simulink model "commhdlQPSKTxRxLoopback"  (R2025b)
settings: Solver=FixedStepDiscrete  StartTime=0.0  StopTime=stopTime  RelTol=1e-3
PostLoadFcn:
  | hScopeConfig = get_param([gcs '/Receiver/QPSK Rx/Frequency and Time Synchronizer/Symbol Synchronizer/No HDL/QPSK Receiver Eye Diagram'],'ScopeConfiguration');
  | 
  | hScopeConfig.OpenAtSimulationStart = false;
  | hScopeConfig.Visible = false;
  | SamplesPerSymbol = 4;
  | %UpsamplesRx = 1;
  | clear hScopeConfig
InitFcn:
  | commhdlQPSKTxRxModelInit;
  | % Rate bridge: ADRV9002/Jupiter radio runs at 15.36 MHz = 2x the 7.68 MHz
  | % (4 samples/symbol @ Rsym=1.92 MHz) the QPSK Rx requires. The deployed
  | % Receiver must downsample the ADC stream by 2. UpsamplesRx=1 fed the QPSK
  | % Rx 8 sps (2x-upsampled) and broke symbol sync / the loopback bit check.
  | UpsamplesRx = 1;   %% T8 RATE FIX: rail 15.36e6 == ADC bus rate,
  | %% no ingress decimation (was 2 when the rail sat on the 7.68e6 rung)
  | UpsamplesTx = 1;
  | clear simTimingOffset;
StopFcn:
  | if exist('simTimingOffset','var')
  |   disp('Simulation completed');
  |   %QPSKTxRxVerification;
  | end
undefined symbols (not defined in the file or in its folder): Add, Config, fsym, randsrc, RandStream, Rsym, Shift
libraries: hdlsllib x141, simulink x43, dspsigops x34, dsphdlfiltering2 x6, dsphdlsigops2 x4, dsphdlmathfun2 x4, commdigbbndpm3 x4, dspmlti4 x2, commchan3 x1, commrflib2 x1, commcnvcod2 x1
(part 3 of 8)

== system commhdlQPSKTxRxLoopback/Receiver/QPSK Rx/Frequency and Time Synchronizer/Coarse Frequency Compensator ==
  dataIn : Inport
  validIn : Inport  Port=2
  CFO step change detector : Subsystem
  Coarse Frequency Estimator : Subsystem
  Data Type Conversion2 : DataTypeConversion  OutDataTypeStr=fixdt(1,16,12)  SaturateOnIntegerOverflow=off  RndMeth=Floor
  Data Type Conversion3 : DataTypeConversion  OutDataTypeStr=fixdt(1,21,21)  SaturateOnIntegerOverflow=off  RndMeth=Floor
  Data Type Conversion4 : DataTypeConversion  OutDataTypeStr=fixdt(1,21,0)  ConvertRealWorld=Stored Integer (SI)  SaturateOnIntegerOverflow=off  RndMeth=Floor
  Delay1 : Delay  DelayLength=9
  Delay{11..17} (7 alike) : Delay
  Delay2 : Delay  DelayLength=9
  Delay3 : Delay  DelayLength=6
  Delay4 : Delay  DelayLength=6
  Delay5 : Delay  DelayLength=1
  Delay6 : Delay  DelayLength=1
  Delay7 : Delay  DelayLength=12
  Delay8 : Delay  DelayLength=12
  Gain : Gain  Gain=1/4  ParamDataTypeStr=fixdt(0,2,2)  OutDataTypeStr=Inherit: Same as input
  Math Function : Math  Operator=conj
  NCO : dsphdlsigops2/NCO  PhaseIncrementSource=Input port  PhaseIncrement=100  PhaseOffsetSource=Property  PhaseOffset=0  DitherSource=None  NumDitherBits=4  SamplesPerFrame=1  LUTCompress=off  ResetAction=off  Waveform=Complex exponential  PhasePort=off  SimulateUsing=Code generation  AccumulatorWL=21  PhaseQuantization=on  NumQuantizerAccumulatorBits=14  OutputDataType=Binary point scaling  OutputWL=16  OutputFL=14
  Product1 : Product  OutDataTypeStr=Inherit: Same as first input
  Raise Power to 4 : Subsystem
  Terminator : Terminator
  dataOut : Outport
  rstCS : Outport  Port=2
  validOut : Outport  Port=3
  normalizedFreqEst : Outport  Port=4
  wires:
  Delay14/1 -> Delay15/1
  Delay11/1 -> Product1/1
  Delay6/1 -> Raise Power to 4/2(validIn), Delay2/1
  Delay5/1 -> Delay1/1, Data Type Conversion2/1
  Data Type Conversion4/1 -> NCO/1
  Delay4/1 -> Delay14/1
  Delay3/1 -> Delay11/1
  Delay2/1 -> Delay8/1
  Delay1/1 -> Delay7/1
  NCO/2 -> Terminator/1
  NCO/1 -> Math Function/1
  Product1/1 -> Delay13/1
  Raise Power to 4/2(validOut) -> Coarse Frequency Estimator/2(validIn)
  Math Function/1 -> Delay12/1
  Raise Power to 4/1(dataOut) -> Coarse Frequency Estimator/1(dataIn)
  Delay12/1 -> Product1/2
  Coarse Frequency Estimator/1(normFreqEst) -> Gain/1
  Data Type Conversion2/1 -> Raise Power to 4/1(dataIn)
  Delay16/1 -> Delay17/1
  CFO step change detector/1(Out1) -> Delay16/1
  Gain/1 -> Data Type Conversion3/1
  Delay13/1 -> dataOut/1
  dataIn/1 -> Delay5/1
  validIn/1 -> Delay6/1
  Delay17/1 -> rstCS/1
  Data Type Conversion3/1 -> normalizedFreqEst/1, CFO step change detector/1(In1), Data Type Conversion4/1
  Delay15/1 -> validOut/1
  Delay7/1 -> Delay3/1
  Delay8/1 -> NCO/2, Delay4/1

== system commhdlQPSKTxRxLoopback/Receiver/QPSK Rx/Frequency and Time Synchronizer/No HDL ==
  In1 : Inport
  In2 : Inport  Port=2
  In3 : Inport  Port=3
  In4 : Inport  Port=4
  Data Type Conversion : DataTypeConversion  OutDataTypeStr=double  SaturateOnIntegerOverflow=off  RndMeth=Floor
  Data Type Conversion1 : DataTypeConversion  OutDataTypeStr=double  SaturateOnIntegerOverflow=off  RndMeth=Floor
  QPSK Receiver Constellations 2 : ConstellationDiagram  NumInputPorts=2  WindowPosition=[67.000000,180.000000,973.000000,678.000000,]  Visible=on  ScopeFrameLocation=window  SymbolsToDisplaySource=Property  SymbolsToDisplay=10000  ReferenceConstellation="{[0.70711+0.70711i        -0.70711+0.70711i        -0.70711-0.70711i         0.70711-0.70711i],[0.70711+0.70711i        -0.70711+0.70711i        -0.70711-0.70711i         0.70711-0.70711i]}"  ReferenceMarker={''+'',''+''}  ReferenceColor={[1 0 0],[1 0 0]}  XLimits=[-1.3581 1.3569]  YLimits=[-1.3581 1.3569]  AxesLimits=[-1.3581 1.3569]  ShowLegend=on  DefaultConfigurationName=comm.scopes.ConstellationDiagramBlockCfg
      settings: OpenAtSimulationStart=off
  Subsystem : Subsystem
  Unit Delay Enabled Synchronous : hdlsllib/Discrete/Unit Delay Enabled Synchronous  InitialCondition=0.0  SampleTime=-1
  Unit Delay Enabled Synchronous1 : hdlsllib/Discrete/Unit Delay Enabled Synchronous  InitialCondition=0.0  SampleTime=-1
  wires:
  In4/1 -> Unit Delay Enabled Synchronous1/2, Subsystem/Enable
  Data Type Conversion/1 -> Unit Delay Enabled Synchronous1/1, Subsystem/1(In1)
  Unit Delay Enabled Synchronous1/1 -> QPSK Receiver Constellations 2/2  "After Carrier Synchronization"
  In2/1 -> Unit Delay Enabled Synchronous/2
  In1/1 -> Data Type Conversion1/1
  Data Type Conversion1/1 -> Unit Delay Enabled Synchronous/1
  Unit Delay Enabled Synchronous/1 -> QPSK Receiver Constellations 2/1  "After Symbol Synchronization"
  In3/1 -> Data Type Conversion/1

== system commhdlQPSKTxRxLoopback/Receiver/QPSK Rx/Frequency and Time Synchronizer/Packet Controller ==
  dataIn : Inport
  syncPulse : Inport  Port=2
  validIn : Inport  Port=3
  Delay : Delay  DelayLength=4
  Delay1 : Delay  DelayLength=4
  Delay2 : Delay  DelayLength=4
  End Generator : Subsystem
  Logical Operator : Logic  IconShape=distinctive  AllPortsSameDT=off  OutDataTypeStr=boolean
  MATLAB Function : MATLAB Function  TreatAsAtomicUnit=on
  Time Scope End Generator : Scope  Commented=on  NumInputPorts=2
      settings: SampleTime=1  ActiveDisplayYMinimum=-0.048155737704917989  ActiveDisplayYMaximum=1.0464480874316939  YLabel=Amplitude  DataLoggingVariableName=ScopeData2
  To File : ToFile  Filename=end_gen.mat  MatrixName=end_gen  SaveFormat=Timeseries
  To File1 : ToFile  Filename=reset  MatrixName=reset  SaveFormat=Timeseries
  sample discard controller : MATLAB Function  TreatAsAtomicUnit=on
  dataOut : Outport
  startOut : Outport  Port=2
  endOut : Outport  Port=3
  validOut : Outport  Port=4
  wires:
  MATLAB Function/1(out) -> Logical Operator/2
  sample discard controller/1(dataOut) -> dataOut/1
  sample discard controller/2(startOut) -> startOut/1
  sample discard controller/3(endOut) -> endOut/1
  sample discard controller/4(validOut) -> validOut/1
  Delay/1 -> sample discard controller/1(dataIn)
  Delay1/1 -> sample discard controller/2(validIn), End Generator/1(validIn)
  Delay2/1 -> sample discard controller/3(startIn)
  dataIn/1 -> Delay/1
  validIn/1 -> MATLAB Function/1(valid), Delay1/1, Logical Operator/1
  Logical Operator/1 -> Delay2/1, To File1/1, Time Scope End Generator/2, End Generator/2(rst)
  syncPulse/1 -> MATLAB Function/2(syncPulse)
  End Generator/1(endOut) -> Time Scope End Generator/1, To File/1, sample discard controller/4(endIn)

== system commhdlQPSKTxRxLoopback/Receiver/QPSK Rx/Frequency and Time Synchronizer/Phase Ambiguity Estimation and Correction ==
  dataIn : Inport
  syncPulseIn : Inport  Port=2
  validIn : Inport  Port=3
  Average Estimates : Subsystem
  Delay : Delay  DelayLength=32
  Delay1 : Delay  DelayLength=32
  Delay10 : Delay  DelayLength=15 + 7
  Delay11 : Delay  DelayLength=5
  Delay12 : Delay  DelayLength=5
  Delay13 : Delay  DelayLength=5
  Delay2 : Delay  DelayLength=32
  Delay3 : Delay  DelayLength=8
  Delay4 : Delay  DelayLength=8
  Delay5 : Delay  DelayLength=8
  Delay6 : Delay  DelayLength=1
  Delay7 : Delay  DelayLength=1
  Delay8 : Delay  DelayLength=1
  Delay9 : Delay  DelayLength=10
  Phase Ambiguity Corrector : Subsystem
  Phase Ambiguity Estimator : Subsystem
  dataOut : Outport
  syncPulseOut : Outport  Port=2
  validOut : Outport  Port=3
  wires:
  Delay4/1 -> Delay2/1
  Delay5/1 -> Delay/1
  Delay3/1 -> Delay1/1
  Delay10/1 -> Delay9/1
  Phase Ambiguity Corrector/1(dataOut) -> dataOut/1
  Phase Ambiguity Corrector/2(validOut) -> validOut/1
  Delay9/1 -> syncPulseOut/1
  Delay8/1 -> Phase Ambiguity Corrector/1(dataIn)
  Average Estimates/1(avgEst) -> Phase Ambiguity Corrector/2(estimate)
  Delay7/1 -> Phase Ambiguity Corrector/3(validIn)
  Delay6/1 -> Delay10/1
  dataIn/1 -> Delay5/1
  validIn/1 -> Delay4/1
  Delay13/1 -> Delay8/1
  Phase Ambiguity Estimator/1(endOut) -> Average Estimates/1(endIn)
  Phase Ambiguity Estimator/3(validOut) -> Average Estimates/3(validIn)
  Delay12/1 -> Delay7/1
  Delay11/1 -> Delay6/1
  Phase Ambiguity Estimator/2(estOut) -> Average Estimates/2(estin)
  Delay/1 -> Delay13/1, Phase Ambiguity Estimator/1(dataIn)
  syncPulseIn/1 -> Phase Ambiguity Estimator/2(syncPulse), Delay3/1
  Delay2/1 -> Phase Ambiguity Estimator/3(validIn), Delay12/1
  Delay1/1 -> Delay11/1

== system commhdlQPSKTxRxLoopback/Receiver/QPSK Rx/Frequency and Time Synchronizer/Preamble Detector ==
  dataIn : Inport
  validIn : Inport  Port=2
  Constant : Constant  Value=false  SampleTime=-1
  Correlator : Subsystem
  Delay : Delay  DelayLength=20
  Delay{1..5,11..14} (9 alike) : Delay  DelayLength=1
  Delay10 : Delay  DelayLength=searchSamples * 4
  Delay6 : Delay  DelayLength=6
  Delay7 : Delay  DelayLength=20
  Delay8 : Delay  DelayLength=6
  FIFO : Subsystem  mask{fifoSize=searchSamples, pushFullDiag=Error, popEmptyDiag=Error}
      mask prompts: fifoSize "FIFO size:"; pushFullDiag "Push full FIFO:"; popEmptyDiag "Pop empty FIFO:"
      mask TypeOptions pushFullDiag: Ignore | Warning | Error
      mask TypeOptions popEmptyDiag: Ignore | Warning | Error
  Logical Operator : Logic  AllPortsSameDT=off  OutDataTypeStr=boolean
  No HDL : Subsystem
  Peak Search : Subsystem  VariantControl=new  mask{samplesPerFrame=searchSamples}
      mask prompts: samplesPerFrame "Number of samples to search:"
      mask init:
      | samplesPerFrame1x            = samplesPerFrame;
      |     searchDuration               = samplesPerFrame1x;
  Relational Operator : RelationalOperator  Operator=>  OutDataTypeStr=boolean  InputSameDT=off
  Terminator : Terminator
  Terminator1 : Terminator
  Timing Adjust : Subsystem
  dataOut : Outport
  syncPulse : Outport  Port=2
  validOut : Outport  Port=3
  wires:
  Delay/1 -> Delay6/1
  validIn/1 -> Delay2/1
  dataIn/1 -> Delay1/1
  Relational Operator/1 -> Peak Search/2(thresholdExceeded)
  Peak Search/3(success) -> Logical Operator/2  "success"
  Peak Search/2(done) -> Logical Operator/1  "done"
  Delay7/1 -> Delay8/1
  Timing Adjust/1(dataOut) -> Delay3/1  "synchronizedData"
  Timing Adjust/3(SyncPulse) -> Delay4/1  "synchronizedPulse"
  Timing Adjust/2(validOut) -> Delay5/1  "synchronizedValid"
  Delay3/1 -> dataOut/1
  Delay5/1 -> validOut/1
  Delay4/1 -> syncPulse/1
  Peak Search/1(timingOffset) -> Delay11/1
  Logical Operator/1 -> Delay12/1
  Delay10/1 -> FIFO/3(pop), Delay14/1
  Correlator/3(validOut) -> Peak Search/3(validIn), No HDL/Enable
  Correlator/2(threshold) -> Relational Operator/2, No HDL/2(In2)
  Correlator/1(dataOut) -> Relational Operator/1, Peak Search/1(corr), No HDL/1(In1)
  Delay8/1 -> FIFO/2(push), Delay10/1
  Delay1/1 -> Delay/1, Correlator/1(dataIn)
  Delay2/1 -> Delay7/1, Correlator/2(validIn)
  Delay11/1 -> Timing Adjust/1(timingOffset)
  Delay12/1 -> Timing Adjust/2(timingOffsetValid)
  Delay13/1 -> Timing Adjust/3(dataIn)
  Delay14/1 -> Timing Adjust/4(validIn)
  FIFO/2(numEntries) -> Terminator/1
  Constant/1 -> FIFO/4(reset)
  FIFO/3(validPop) -> Terminator1/1
  Delay6/1 -> FIFO/1(in)
  FIFO/1(out) -> Delay13/1

== system commhdlQPSKTxRxLoopback/Receiver/QPSK Rx/Frequency and Time Synchronizer/Symbol Synchronizer ==
  dataIn : Inport
  validIn : Inport  Port=2
  Data Type Conversion4 : DataTypeConversion  OutDataTypeStr=fixdt(1,16,14)  SaturateOnIntegerOverflow=off  RndMeth=Floor
  Delay{1..4,6,8..9} (7 alike) : Delay  DelayLength=1
  Delay5 : Delay  DelayLength=12
  Delay7 : Delay  DelayLength=12
  Gardner TED : Subsystem
  Integer Delay{1..4} (4 alike) : Delay  DelayLength=1
  Interpolation Control : MATLAB Function
  Interpolation Filter : Subsystem
  Loop Filter : Subsystem
  No HDL : Subsystem
  Rate Handle : Subsystem
  dataOut : Outport
  validOut : Outport  Port=2
  wires:
  Loop Filter/1(v) -> Delay4/1
  Gardner TED/1(e) -> Delay3/1
  Interpolation Control/2(Underflow) -> Integer Delay3/1
  Integer Delay4/1 -> Interpolation Filter/2(mu)
  dataIn/1 -> No HDL/1(data), Integer Delay1/1
  Integer Delay3/1 -> Delay5/1
  Delay3/1 -> Loop Filter/1(e)
  Delay4/1 -> Interpolation Control/1(Delta)
  Data Type Conversion4/1 -> Rate Handle/1(dataIn)
  Delay1/1 -> Data Type Conversion4/1
  Delay6/1 -> Rate Handle/3(validIn)
  Delay7/1 -> Delay6/1
  validIn/1 -> No HDL/2(valid), Integer Delay2/1
  Rate Handle/2(validOut) -> validOut/1
  Rate Handle/1(dataOut) -> dataOut/1
  Interpolation Filter/1(interpolant) -> Delay8/1, Delay1/1
  Interpolation Control/1(mu) -> Integer Delay4/1
  Delay2/1 -> Rate Handle/2(strobe)
  Delay5/1 -> Delay9/1, Delay2/1
  Integer Delay1/1 -> Interpolation Filter/1(In)
  Integer Delay2/1 -> Delay7/1
  Delay8/1 -> Gardner TED/1(data)
  Delay9/1 -> Gardner TED/2(strobe)

== system commhdlQPSKTxRxLoopback/Receiver/QPSK Rx/QPSK Demodulator/Serializer ==
  u : Inport
  In2 : Inport  Port=2
  Delay1 : Delay  DelayLength=1
  Delay4 : Delay  DelayLength=1
  Demux : Demux  Outputs=2
  HDL Counter : hdlsllib/Sources/HDL Counter  CountType=Count limited  CountInit=0  CountStep=1  CountMax=1  CountFromType=Initial value  CountFrom=0  CountResetPort=off  CountLoadPort=off  CountEnbPort=on  CountDirPort=off  CountHitOutputPort=off  CountDataType=Unsigned  CountWordLen=1  CountFracLen=0  CountSampTime=1
  Logical Operator : Logic  Operator=OR  AllPortsSameDT=off  OutDataTypeStr=boolean
  Multiport Switch : MultiPortSwitch  DataPortOrder=Zero-based contiguous  Inputs=2  zeroidx=on  SaturateOnIntegerOverflow=off  InputSameDT=off
  Unit Delay Enabled Synchronous : hdlsllib/Discrete/Unit Delay Enabled Synchronous  InitialCondition=0.0  SampleTime=-1
  Out1 : Outport
  Out2 : Outport  Port=2
  wires:
  Demux/2 -> Multiport Switch/3
  Logical Operator/1 -> Out2/1, HDL Counter/1
  In2/1 -> Unit Delay Enabled Synchronous/2, Delay1/1
  HDL Counter/1 -> Multiport Switch/1
  Delay4/1 -> Logical Operator/2
  u/1 -> Unit Delay Enabled Synchronous/1
  Multiport Switch/1 -> Out1/1
  Demux/1 -> Multiport Switch/2
  Delay1/1 -> Logical Operator/1, Delay4/1
  Unit Delay Enabled Synchronous/1 -> Demux/1

== system commhdlQPSKTxRxLoopback/Transmitter/QPSK Tx/Bit Packetizer/Data Bits FIFO ==
  data : Inport
  push : Inport  Port=2
  Compare To Constant : simulink/Logic and Bit Operations/Compare To Constant  relop=>=  const=length(Preamble)  OutDataTypeStr=boolean
  Compare To Constant1 : simulink/Logic and Bit Operations/Compare To Constant  relop===  const=0  OutDataTypeStr=boolean
  Compare To Constant2 : simulink/Logic and Bit Operations/Compare To Constant  relop=~=  const=0  OutDataTypeStr=boolean
  Compare To Constant3 : simulink/Logic and Bit Operations/Compare To Constant  relop===  const=0  OutDataTypeStr=boolean
  Compare To Constant4 : simulink/Logic and Bit Operations/Compare To Constant  relop===  const=bitsPerPacket - 1  OutDataTypeStr=boolean
  Compare To Constant5 : hdlsllib/Logic and Bit Operations/Compare To Constant  relop===  const=Config.SamplesPerSymbol/2 -1  OutDataTypeStr=boolean
  Constant : Constant  Value=true  SampleTime=1/(Rsym*SamplesPerSymbol)
  Delay{1..7} (7 alike) : Delay  DelayLength=1
  HDL Counter : hdlsllib/Sources/HDL Counter  CountType=Count limited  CountInit=0  CountStep=1  CountMax=dataBitsPerPacket*2 - 1  CountFromType=Initial value  CountFrom=0  CountResetPort=off  CountLoadPort=off  CountEnbPort=on  CountDirPort=off  CountHitOutputPort=off  CountDataType=Unsigned  CountWordLen=nextpow2(dataBitsPerPacket*2 - 1)  CountFracLen=0  CountSampTime=1
  HDL Counter1 : hdlsllib/Sources/HDL Counter  CountType=Count limited  CountInit=0  CountStep=1  CountMax=dataBitsPerPacket*2 - 1  CountFromType=Initial value  CountFrom=0  CountResetPort=off  CountLoadPort=off  CountEnbPort=on  CountDirPort=off  CountHitOutputPort=off  CountDataType=Unsigned  CountWordLen=nextpow2(dataBitsPerPacket*2 - 1)  CountFracLen=0  CountSampTime=1
  HDL Counter2 : hdlsllib/Sources/HDL Counter  CountType=Count limited  CountInit=0  CountStep=1  CountMax=bitsPerPacket - 1  CountFromType=Initial value  CountFrom=0  CountResetPort=off  CountLoadPort=off  CountEnbPort=on  CountDirPort=off  CountHitOutputPort=off  CountDataType=Unsigned  CountWordLen=nextpow2(bitsPerPacket)  CountFracLen=0  CountSampTime=1
  HDL Counter3 : hdlsllib/Sources/HDL Counter  CountType=Count limited  CountInit=0  CountStep=1  CountMax=Config.SamplesPerSymbol/2 -1  CountFromType=Initial value  CountFrom=0  CountResetPort=off  CountLoadPort=off  CountEnbPort=on  CountDirPort=off  CountHitOutputPort=off  CountDataType=Unsigned  CountWordLen=nextpow2(Config.SamplesPerSymbol/2)  CountFracLen=0  CountSampTime=1
  Logical Operator : Logic  Inputs=3  AllPortsSameDT=off  OutDataTypeStr=boolean
  Logical Operator1 : Logic  Inputs=3  AllPortsSameDT=off  OutDataTypeStr=boolean
  MATLAB Function1 : MATLAB Function  TreatAsAtomicUnit=on
  No HDL : Subsystem
  RAM Frame Status Indicator : MATLAB Function  TreatAsAtomicUnit=on
  Simple Dual Port RAM : hdlsllib/HDL RAMs/Simple Dual Port RAM  ram_size=nextpow2(dataBitsPerPacket*2 - 1)
  Unit Delay Enabled Resettable Synchronous : hdlsllib/Discrete/Unit Delay Enabled Resettable Synchronous  InitialCondition=0.0  SampleTime=-1
  dataOut : Outport
  activeFrame : Outport  Port=2
  sampleCount : Outport  Port=3
  sampleCountValid : Outport  Port=4
  fullRAM : Outport  Port=5
  wires:
  HDL Counter1/1 -> Simple Dual Port RAM/4
  HDL Counter/1 -> Simple Dual Port RAM/2
  data/1 -> Simple Dual Port RAM/1
  Constant/1 -> HDL Counter3/1
  HDL Counter2/1 -> Compare To Constant/1, Delay2/1, Compare To Constant3/1
  Compare To Constant1/1 -> Unit Delay Enabled Resettable Synchronous/3
  RAM Frame Status Indicator/1(out) -> Delay3/1
  Compare To Constant2/1 -> Logical Operator1/1, Unit Delay Enabled Resettable Synchronous/1
  Compare To Constant3/1 -> Unit Delay Enabled Resettable Synchronous/2
  Compare To Constant/1 -> Delay1/1
  Delay1/1 -> Logical Operator/2
  Delay2/1 -> Delay5/1
  Delay3/1 -> Compare To Constant2/1, Compare To Constant1/1
  Simple Dual Port RAM/1 -> dataOut/1
  Delay4/1 -> Logical Operator/3, Delay6/1
  Delay5/1 -> Compare To Constant4/1, sampleCount/1
  Delay6/1 -> Logical Operator1/3, sampleCountValid/1
  Unit Delay Enabled Resettable Synchronous/1 -> Logical Operator/1
  Compare To Constant4/1 -> Logical Operator1/2
  Logical Operator1/1 -> activeFrame/1
  Logical Operator/1 -> RAM Frame Status Indicator/2(pop), MATLAB Function1/2(rd), No HDL/2(pop), HDL Counter1/1
  push/1 -> MATLAB Function1/1(wr), RAM Frame Status Indicator/1(push), No HDL/1(push), HDL Counter/1, Simple Dual Port RAM/3
  MATLAB Function1/1(full) -> Delay7/1
  Delay7/1 -> fullRAM/1
  HDL Counter3/1 -> Compare To Constant5/1
  Compare To Constant5/1 -> HDL Counter2/1, Delay4/1

== system commhdlQPSKTxRxLoopback/Transmitter/QPSK Tx/Bit Packetizer/Preamble Bits Generator ==
  activeFrame : Inport
  sampleCount : Inport  Port=2
  sampleCountValid : Inport  Port=3
  Compare To Constant2 : hdlsllib/Logic and Bit Operations/Compare To Constant  relop===  const=bitsPerPacket - 1  OutDataTypeStr=boolean
  Logical Operator3 : Logic  AllPortsSameDT=off  OutDataTypeStr=boolean
  Preamble Bits Store : Subsystem
  Unit Delay Enabled Synchronous : hdlsllib/Discrete/Unit Delay Enabled Synchronous  InitialCondition=0.0  SampleTime=-1
  preambleBits : Outport
  wires:
  sampleCount/1 -> Compare To Constant2/1, Preamble Bits Store/2(sampleCount)
  Logical Operator3/1 -> Unit Delay Enabled Synchronous/2
  Preamble Bits Store/1(preamble) -> preambleBits/1
  Compare To Constant2/1 -> Logical Operator3/1
  Unit Delay Enabled Synchronous/1 -> Preamble Bits Store/1(actualPreamble)
  sampleCountValid/1 -> Logical Operator3/2
  activeFrame/1 -> Unit Delay Enabled Synchronous/1

== system commhdlQPSKTxRxLoopback/TxRxComposite/Receiver/QPSK Rx/Automatic Gain Control ==
  dataIn : Inport
  validIn : Inport  Port=2
  agc_loop_gain : Inport  Port=3  OutDataTypeStr=uint32  SampleTime=1/(Rsym*SamplesPerSymbol)
  Data Type Conversion : DataTypeConversion  OutDataTypeStr=fixdt(1,16,10)  SaturateOnIntegerOverflow=off  RndMeth=Floor
  Delay{1..5} (5 alike) : Delay
  Error Detector : Subsystem
  Loop Filter : Subsystem
  Product : Product  OutDataTypeStr=Inherit: Same as first input
  dataOut : Outport
  validOut : Outport  Port=2
  wires:
  Product/1 -> Delay2/1
  dataIn/1 -> Delay4/1
  Delay2/1 -> dataOut/1, Error Detector/1(dataIn)
  validIn/1 -> Delay5/1
  Error Detector/1(err) -> Loop Filter/1(err)
  Loop Filter/1(gain) -> Data Type Conversion/1
  Delay1/1 -> Product/2
  Delay4/1 -> Product/1
  Delay3/1 -> validOut/1
  Delay5/1 -> Delay3/1
  Data Type Conversion/1 -> Delay1/1
  agc_loop_gain/1 -> Loop Filter/2(agc_loop_gain)

== system commhdlQPSKTxRxLoopback/TxRxComposite/Receiver/QPSK Rx/FEC Decoder Wrapper ==
  bitsIn : Inport
  startIn : Inport  Port=2
  endIn : Inport  Port=3
  validIn : Inport  Port=4
  skipCount : Inport  Port=5  OutDataTypeStr=uint32  SampleTime=1/(Rsym*SamplesPerSymbol)
  FecCapture : MATLAB Function  TreatAsAtomicUnit=on
  FecCounters : MATLAB Function  TreatAsAtomicUnit=on
  RxAlign : MATLAB Function  TreatAsAtomicUnit=on
  RxDeint : MATLAB Function  TreatAsAtomicUnit=on
  VitGate : Subsystem
  dataOut : Outport
  startOut : Outport  Port=2
  endOut : Outport  Port=3
  validOut : Outport  Port=4
  cnt_descr_in : Outport  Port=5
  cnt_frame_start : Outport  Port=6
  cnt_vit_reset : Outport  Port=7
  cnt_deint_valid : Outport  Port=8
  cnt_dec_bits : Outport  Port=9
  cnt_bist_start : Outport  Port=10
  cap_in : Outport  Port=11
  cap_deint : Outport  Port=12
  cap_out : Outport  Port=13
  wires:
  bitsIn/1 -> RxDeint/1(dataIn), FecCapture/1(bitsIn)
  startIn/1 -> RxDeint/2(startIn), FecCounters/2(e2), FecCapture/3(startIn)
  endIn/1 -> RxDeint/3(endIn)
  validIn/1 -> RxDeint/4(validIn), FecCounters/1(e1), FecCapture/2(validIn)
  RxDeint/1(codedPair) -> VitGate/1(pairIn), FecCapture/4(codedPair)
  RxDeint/2(vitReset) -> VitGate/2(rstIn), FecCounters/3(e3)
  RxDeint/3(deintValid) -> VitGate/Enable, RxAlign/2(deintValid), FecCounters/4(e4), FecCapture/5(deintValid)
  VitGate/1(decOut) -> RxAlign/1(decBit)
  RxDeint/4(frameStart) -> RxAlign/3(frameStart)
  RxDeint/5(frameEnd) -> RxAlign/4(frameEnd)
  skipCount/1 -> RxAlign/5(skipCount), FecCapture/7(skipCount)
  RxAlign/1(dataOut) -> dataOut/1, FecCapture/6(decBit)
  RxAlign/2(startOut) -> startOut/1, FecCounters/6(e6)
  RxAlign/3(endOut) -> endOut/1
  RxAlign/4(validOut) -> validOut/1, FecCounters/5(e5), FecCapture/8(outValid)
  FecCounters/1(c1) -> cnt_descr_in/1
  FecCounters/2(c2) -> cnt_frame_start/1
  FecCounters/3(c3) -> cnt_vit_reset/1
  FecCounters/4(c4) -> cnt_deint_valid/1
  FecCounters/5(c5) -> cnt_dec_bits/1
  FecCounters/6(c6) -> cnt_bist_start/1
  FecCapture/1(capIn) -> cap_in/1
  FecCapture/2(capDeint) -> cap_deint/1
  FecCapture/3(capOut) -> cap_out/1

== system commhdlQPSKTxRxLoopback/TxRxComposite/Receiver/QPSK Rx/Frequency and Time Synchronizer ==
  dataIn : Inport
  validIn : Inport  Port=2
  rstCS : Inport  Port=3
  cs_prop_gain : Inport  Port=4  OutDataTypeStr=uint32  SampleTime=1/(Rsym*SamplesPerSymbol)
  cs_integ_gain : Inport  Port=5  OutDataTypeStr=uint32  SampleTime=1/(Rsym*SamplesPerSymbol)
  ss_prop_gain : Inport  Port=6  OutDataTypeStr=uint32  SampleTime=1/(Rsym*SamplesPerSymbol)
  ss_integ_gain : Inport  Port=7  OutDataTypeStr=uint32  SampleTime=1/(Rsym*SamplesPerSymbol)
  cfo_threshold : Inport  Port=8  OutDataTypeStr=uint32  SampleTime=1/(Rsym*SamplesPerSymbol)
  Carrier Synchronizer : Subsystem
      settings: PortSchema="{\"entries\":[{\"content\":{\"sides\":[{\"content\":{\"connectorIds\":[\"In1\",\"In2\",\"In3\"]},\"type\":\"ConnectorPlacement.EquallySpacedRectSide\",\"uuid\":\"ee58e5dc-083a-48cb-b7f3-66ed8a15890f\"},{\"content\":{\"connectorIds\":[\"Out1\",\"Out2\"],\"side\":\"RIGHT\"},\"type\":\"ConnectorPlacement.EquallySpacedRectSide\",\"uuid\":\"6d121164-5065-4840-a82e-fa57a8e9650e\"},{\"content\":{\"connectorIds\":[\"In4\",\"In5\",\"In6\"],\"side\":\"TOP\"},\"type\":\"ConnectorPlacement.EquallySpacedRectSide\",\"uuid\":\"54d2b8e3-f516-4572-94a0-c914196ae8e4\"}]},\"type\":\"ConnectorPlacement.EquallySpacedConnector\",\"uuid\":\"0f2a6472-efd0-42ca-a030-ab436081b5e1\"}],\"packageUris\":[\"http://schema.mathworks.com/mf0/Connector/R2020b\"],\"version\":\"1.0\"}"
  Coarse Frequency Compensator : Subsystem
      settings: PortSchema="{\"entries\":[{\"content\":{\"sides\":[{\"content\":{\"connectorIds\":[\"In1\",\"In2\",\"In3\"]},\"type\":\"ConnectorPlacement.EquallySpacedRectSide\",\"uuid\":\"138aa5bd-62db-47d6-b55f-f529a6004434\"},{\"content\":{\"connectorIds\":[\"Out1\",\"Out2\",\"Out3\"],\"side\":\"RIGHT\"},\"type\":\"ConnectorPlacement.EquallySpacedRectSide\",\"uuid\":\"8e6ccec0-f736-48ab-be6d-feac886e083d\"},{\"content\":{\"connectorIds\":[\"Out4\"],\"side\":\"TOP\"},\"type\":\"ConnectorPlacement.EquallySpacedRectSide\",\"uuid\":\"d4535392-74fa-432a-a39c-b98ba26e8163\"},{\"content\":{\"side\":\"BOTTOM\"},\"type\":\"ConnectorPlacement.EquallySpacedRectSide\",\"uuid\":\"770ac6a2-7a02-4a77-858b-592982deaf6e\"}]},\"type\":\"ConnectorPlacement.EquallySpacedConnector\",\"uuid\":\"a9b944be-f88b-4ab6-a5e1-6824362eb9ca\"}],\"packageUris\":[\"http://schema.mathworks.com/mf0/Connector/R2020b\"],\"version\":\"1.0\"}"
  No HDL : Subsystem
      settings: PortSchema="{\"entries\":[{\"content\":{\"sides\":[{\"content\":{\"connectorIds\":[\"In1\",\"In2\"]},\"type\":\"ConnectorPlacement.EquallySpacedRectSide\",\"uuid\":\"df96a46d-149f-4580-adf6-e5cf26cffa9b\"},{\"content\":{\"connectorIds\":[\"In3\",\"In4\"],\"side\":\"RIGHT\"},\"type\":\"ConnectorPlacement.EquallySpacedRectSide\",\"uuid\":\"1c46d09c-cb37-4618-ac4e-e5ef50df41fb\"},{\"content\":{\"connectorIds\":[],\"side\":\"TOP\"},\"type\":\"ConnectorPlacement.EquallySpacedRectSide\",\"uuid\":\"7fe62300-46d7-4234-a31d-eecffed4f6e6\"},{\"content\":{\"connectorIds\":[],\"side\":\"BOTTOM\"},\"type\":\"ConnectorPlacement.EquallySpacedRectSide\",\"uuid\":\"05ecd563-28f5-4cfd-b718-5032a7458763\"}]},\"type\":\"ConnectorPlacement.EquallySpacedConnector\",\"uuid\":\"4b3d5859-a469-4389-9e5d-e5f07416a9a1\"}],\"packageUris\":[\"http://schema.mathworks.com/mf0/Connector/R2020b\"],\"version\":\"1.0\"}"
  Packet Controller : Subsystem
  Phase Ambiguity Estimation and Correction : Subsystem
  Preamble Detector : Subsystem
  Symbol Synchronizer : Subsystem
  dataOut : Outport
  startOut : Outport  Port=2
  endOut : Outport  Port=3
  validOut : Outport  Port=4
  postSymbolSync : Outport  Port=5
  postCarrierSync : Outport  Port=6
  nSynced : Outport  Port=7
  normCoarseFreqEst : Outport  Port=8
  rstcsDet : Outport  Port=9
  p1c_telI : Outport  Port=10
  p1c_telQ : Outport  Port=11
  fs_runmax : Outport  Port=12
  wires:
  rstCS/1 -> Carrier Synchronizer/4(manualRst)
  Coarse Frequency Compensator/4(normalizedFreqEst) -> normCoarseFreqEst/1
  Carrier Synchronizer/2(validOut) -> Preamble Detector/2(validIn), No HDL/4(In4)
  Carrier Synchronizer/1(dataOut) -> Preamble Detector/1(dataIn), No HDL/3(In3), postCarrierSync/1
  Preamble Detector/2(syncPulse) -> Phase Ambiguity Estimation and Correction/2(syncPulseIn), nSynced/1
  Packet Controller/4(validOut) -> validOut/1
  Packet Controller/3(endOut) -> endOut/1
  Packet Controller/2(startOut) -> startOut/1
  Packet Controller/1(dataOut) -> dataOut/1
  Coarse Frequency Compensator/2(rstCS) -> Carrier Synchronizer/2(internalRst), rstcsDet/1
  dataIn/1 -> Symbol Synchronizer/1(dataIn)
  validIn/1 -> Symbol Synchronizer/2(validIn)
  Preamble Detector/1(dataOut) -> Phase Ambiguity Estimation and Correction/1(dataIn)
  Preamble Detector/3(validOut) -> Phase Ambiguity Estimation and Correction/3(validIn)
  Phase Ambiguity Estimation and Correction/2(syncPulseOut) -> Packet Controller/2(syncPulse)
  Symbol Synchronizer/1(dataOut) -> Coarse Frequency Compensator/1(dataIn), No HDL/1(In1), postSymbolSync/1
  Symbol Synchronizer/2(validOut) -> Coarse Frequency Compensator/2(validIn), No HDL/2(In2)
  Phase Ambiguity Estimation and Correction/3(validOut) -> Packet Controller/3(validIn)
  Phase Ambiguity Estimation and Correction/1(dataOut) -> Packet Controller/1(dataIn)
  Coarse Frequency Compensator/1(dataOut) -> Carrier Synchronizer/1(dataIn)
  Coarse Frequency Compensator/3(validOut) -> Carrier Synchronizer/3(validIn)
  Preamble Detector/4(p1c_telI) -> p1c_telI/1
  Preamble Detector/5(p1c_telQ) -> p1c_telQ/1
  cs_prop_gain/1 -> Carrier Synchronizer/5(cs_prop_gain)
  cs_integ_gain/1 -> Carrier Synchronizer/6(cs_integ_gain)
  ss_prop_gain/1 -> Symbol Synchronizer/3(ss_prop_gain)
  ss_integ_gain/1 -> Symbol Synchronizer/4(ss_integ_gain)
  cfo_threshold/1 -> Coarse Frequency Compensator/3(cfo_threshold)
  Preamble Detector/6(fs_runmax) -> fs_runmax/1

== system commhdlQPSKTxRxLoopback/TxRxComposite/Receiver/QPSK Rx/QPSK Demodulator ==
  dataIn : Inport
  startIn : Inport  Port=2
  endIn : Inport  Port=3
  validIn : Inport  Port=4
  Delay{,1..13} (14 alike) : Delay  DelayLength=1
  QPSK Demodulator Baseband : commdigbbndpm3/QPSK Demodulator Baseband  OutType=Bit  DecType=Hard decision  VarSource=Dialog  Variance=1  Dec=Gray  Ph=pi/4  outDtype1=boolean  outDtype2=Inherit via internal rule  derotateFactorWordLen=16  derotateFactorDataTypeStr=Inherit: Same word length as input  derotateFactorLastDataTypeStr=Inherit: Same word length as input
  Serializer : Subsystem
  Signal Specification : SignalSpecification  Dimensions=1
  dataOut : Outport
  startOut : Outport  Port=2
  endOut : Outport  Port=3
  validOut : Outport  Port=4
  wires:
  endIn/1 -> Delay3/1
  startIn/1 -> Delay2/1
  validIn/1 -> Delay1/1
  dataIn/1 -> Signal Specification/1
  Serializer/2(Out2) -> Delay9/1
  Serializer/1(Out1) -> Delay8/1
  Delay13/1 -> Delay11/1
  Delay4/1 -> Delay10/1
  Delay12/1 -> Serializer/1(u)
  Delay5/1 -> Serializer/2(In2)
  Delay11/1 -> endOut/1
  Delay10/1 -> startOut/1
  Delay9/1 -> validOut/1
  Delay8/1 -> dataOut/1
  QPSK Demodulator Baseband/1 -> Delay12/1
  Signal Specification/1 -> Delay/1
  Delay3/1 -> Delay7/1
  Delay2/1 -> Delay6/1
  Delay7/1 -> Delay13/1
  Delay6/1 -> Delay4/1
  Delay1/1 -> Delay5/1
  Delay/1 -> QPSK Demodulator Baseband/1

== system commhdlQPSKTxRxLoopback/TxRxComposite/Transmitter/Input Data/FEC Tx Encoder K5 ==
  bitIn : Inport
  enable : Inport  Port=2
  reset : Inport  Port=3
  start : Inport  Port=4
  ConvEncK5 : MATLAB Function  TreatAsAtomicUnit=on
  TxGateK5 : MATLAB Function  TreatAsAtomicUnit=on
  TxInterleaveK5 : MATLAB Function  TreatAsAtomicUnit=on
  encBit : Outport
  wires:
  bitIn/1 -> TxGateK5/1(bitIn)
  enable/1 -> TxGateK5/2(enable)
  reset/1 -> TxGateK5/3(reset)
  start/1 -> TxGateK5/4(start)
  TxGateK5/1(infoBit) -> ConvEncK5/1(infoBit)
  TxGateK5/2(encReset) -> ConvEncK5/2(encReset)
  TxGateK5/3(infoValid) -> ConvEncK5/3(infoValid), TxInterleaveK5/2(infoValid)
  ConvEncK5/1(codedPair) -> TxInterleaveK5/1(codedPair)
  TxGateK5/4(beatIdx) -> TxInterleaveK5/3(beatIdx)
  TxGateK5/5(frameValid) -> TxInterleaveK5/4(frameValid)
  TxGateK5/6(frameStart) -> TxInterleaveK5/5(frameStart)
  TxInterleaveK5/1(dataOut) -> encBit/1

== system commhdlQPSKTxRxLoopback/TxRxComposite/Transmitter/Input Data/Message Generator ==
  reset : Inport
  enable : Inport  Port=2
  MATLAB Function : MATLAB Function  TreatAsAtomicUnit=on
  out : Outport
  stop : Outport  Port=2
  start : Outport  Port=3
  valid : Outport  Port=4
  count : Outport  Port=5
  msg_count_out : Outport  Port=6
  wires:
  MATLAB Function/6(msg_count_out) -> msg_count_out/1
  MATLAB Function/5(count_out) -> count/1
  MATLAB Function/4(valid) -> valid/1
  enable/1 -> MATLAB Function/1(enable)
  MATLAB Function/2(start) -> start/1
  reset/1 -> MATLAB Function/2(reset)
  MATLAB Function/1(out) -> out/1
  MATLAB Function/3(stop) -> stop/1

== system commhdlQPSKTxRxLoopback/TxRxComposite/Transmitter/QPSK Tx/Bit Packetizer ==
  dataIn : Inport
  validIn : Inport  Port=2
  Compare To Constant : hdlsllib/Logic and Bit Operations/Compare To Constant  relop===  const=length(Preamble)  OutDataTypeStr=boolean
  Compare To Constant1 : hdlsllib/Logic and Bit Operations/Compare To Constant  relop===  const=bitsPerPacket - 1  OutDataTypeStr=boolean
  Compare To Constant2 : hdlsllib/Logic and Bit Operations/Compare To Constant  relop=>=  const=length(Preamble)  OutDataTypeStr=boolean
  Data Bits FIFO : Subsystem
  Data Type Conversion : DataTypeConversion  OutDataTypeStr=boolean  SaturateOnIntegerOverflow=off  RndMeth=Floor
  DataReadyPaceCmp : simulink/Logic and Bit Operations/Compare To Constant  relop===  const=SamplesPerSymbol/2 - 1  OutDataTypeStr=boolean
  HDL Counter : hdlsllib/Sources/HDL Counter  CountType=Count limited  CountInit=0  CountStep=1  CountMax=SamplesPerSymbol/2 - 1  CountFromType=Initial value  CountFrom=0  CountResetPort=off  CountLoadPort=off  CountEnbPort=on  CountDirPort=off  CountHitOutputPort=off  CountDataType=Unsigned  CountWordLen=nextpow2(SamplesPerSymbol/2)  CountFracLen=0  CountSampTime=1
  Logical Operator : Logic  AllPortsSameDT=off  OutDataTypeStr=boolean
  Logical Operator1 : Logic  AllPortsSameDT=off  OutDataTypeStr=boolean
  Logical Operator2 : Logic  Operator=NOT  AllPortsSameDT=off  OutDataTypeStr=boolean
  Preamble Bits Generator : Subsystem
  Switch : Switch  Criteria=u2 ~= 0  SaturateOnIntegerOverflow=off  InputSameDT=off
  bitsOut : Outport
  dataStart : Outport  Port=2
  dataEnd : Outport  Port=3
  bitsValid : Outport  Port=4
  dataReady : Outport  Port=5
  wires:
  DataReadyPaceCmp/1 -> Data Type Conversion/1
  HDL Counter/1 -> DataReadyPaceCmp/1
  Data Type Conversion/1 -> dataReady/1
  Switch/1 -> bitsOut/1
  Compare To Constant2/1 -> Switch/2
  Preamble Bits Generator/1(preambleBits) -> Switch/3
  Data Bits FIFO/2(activeFrame) -> Preamble Bits Generator/1(activeFrame)
  Data Bits FIFO/4(sampleCountValid) -> Preamble Bits Generator/3(sampleCountValid), Logical Operator1/1, Logical Operator/2, bitsValid/1
  Data Bits FIFO/3(sampleCount) -> Compare To Constant2/1, Compare To Constant1/1, Compare To Constant/1, Preamble Bits Generator/2(sampleCount)
  Data Bits FIFO/1(dataOut) -> Switch/1
  Logical Operator2/1 -> HDL Counter/1
  Data Bits FIFO/5(fullRAM) -> Logical Operator2/1
  Logical Operator1/1 -> dataEnd/1
  Logical Operator/1 -> dataStart/1
  Compare To Constant1/1 -> Logical Operator1/2
  Compare To Constant/1 -> Logical Operator/1
  validIn/1 -> Data Bits FIFO/2(push)
  dataIn/1 -> Data Bits FIFO/1(data)

== system commhdlQPSKTxRxLoopback/TxRxComposite/Transmitter/QPSK Tx/HDL Data Scrambler ==
  note: HDL Data Scrambler
      | Polynomial: x^7+x^4+1
      | Initial state: [1 0 1 1 1 0 1]
  dataIn : Inport
  startIn : Inport  Port=2
  endIn : Inport  Port=3
  validIn : Inport  Port=4
  BIT_XOR : Logic  Operator=XOR  IconShape=distinctive  AllPortsSameDT=off  OutDataTypeStr=boolean
  BIT_XOR2 : Logic  Operator=XOR  IconShape=distinctive  AllPortsSameDT=off  OutDataTypeStr=boolean
  Delay{,1,3..4} (4 alike) : Delay  DelayLength=1
  EnableScrambling : Constant  Value=false  SampleTime=-1
  Logical Operator : Logic  IconShape=distinctive  AllPortsSameDT=off  OutDataTypeStr=boolean
  Switch : Switch  Criteria=u2 > Threshold  SaturateOnIntegerOverflow=off  InputSameDT=off
  Unit Delay Enabled Resettable Synchronous{,2..3,5,7} (5 alike) : hdlsllib/Discrete/Unit Delay Enabled Resettable Synchronous  InitialCondition=1  SampleTime=-1
  Unit Delay Enabled Resettable Synchronous1 : hdlsllib/Discrete/Unit Delay Enabled Resettable Synchronous  InitialCondition=0  SampleTime=-1
  Unit Delay Enabled Resettable Synchronous4 : hdlsllib/Discrete/Unit Delay Enabled Resettable Synchronous  InitialCondition=0  SampleTime=-1
  Unit Delay Enabled Resettable Synchronous6 : hdlsllib/Discrete/Unit Delay Enabled Resettable Synchronous  InitialCondition=0.0  SampleTime=-1
  dataOut : Outport  InitialOutput=0
  validOut : Outport  Port=2  InitialOutput=0
  wires:
  BIT_XOR2/1 -> Switch/1
  EnableScrambling/1 -> Switch/2
  Switch/1 -> Delay3/1
  Unit Delay Enabled Resettable Synchronous7/1 -> BIT_XOR/1
  Unit Delay Enabled Resettable Synchronous6/1 -> Unit Delay Enabled Resettable Synchronous7/1
  Unit Delay Enabled Resettable Synchronous5/1 -> Unit Delay Enabled Resettable Synchronous6/1
  Unit Delay Enabled Resettable Synchronous3/1 -> Unit Delay Enabled Resettable Synchronous5/1, BIT_XOR/2
  Unit Delay Enabled Resettable Synchronous/1 -> Unit Delay Enabled Resettable Synchronous1/1
  Unit Delay Enabled Resettable Synchronous2/1 -> Unit Delay Enabled Resettable Synchronous3/1
  Unit Delay Enabled Resettable Synchronous1/1 -> Unit Delay Enabled Resettable Synchronous2/1
  BIT_XOR/1 -> Logical Operator/2, Unit Delay Enabled Resettable Synchronous/1
  validIn/1 -> Delay1/1
  dataIn/1 -> Delay/1
  startIn/1 -> Unit Delay Enabled Resettable Synchronous7/3, Unit Delay Enabled Resettable Synchronous3/3, Unit Delay Enabled Resettable Synchronous2/3, Unit Delay Enabled Resettable Synchronous/3, Unit Delay Enabled Resettable Synchronous1/3, Unit Delay Enabled Resettable Synchronous5/3, Unit Delay Enabled Resettable Synchronous6/3, Unit Delay Enabled Resettable Synchronous4/2, Unit Delay Enabled Resettable Synchronous4/1
  Delay/1 -> BIT_XOR2/1, Switch/3
  Delay1/1 -> Unit Delay Enabled Resettable Synchronous7/2, Unit Delay Enabled Resettable Synchronous5/2, Unit Delay Enabled Resettable Synchronous3/2, Delay4/1, Unit Delay Enabled Resettable Synchronous/2, Unit Delay Enabled Resettable Synchronous1/2, Unit Delay Enabled Resettable Synchronous2/2, Unit Delay Enabled Resettable Synchronous6/2
  Unit Delay Enabled Resettable Synchronous4/1 -> Logical Operator/1
  Logical Operator/1 -> BIT_XOR2/2
  endIn/1 -> Unit Delay Enabled Resettable Synchronous4/3
  Delay3/1 -> dataOut/1
  Delay4/1 -> validOut/1

== system commhdlQPSKTxRxLoopback/TxRxComposite/Transmitter/QPSK Tx/QPSK Modulator ==
  dataIn : Inport
  validIn : Inport  Port=2
  Compare To Constant : simulink/Logic and Bit Operations/Compare To Constant  relop===  const=0  OutDataTypeStr=boolean
  Compare To Constant1 : simulink/Logic and Bit Operations/Compare To Constant  relop===  const=1  OutDataTypeStr=boolean
  Delay{,1..5,11..12} (8 alike) : Delay  DelayLength=1
  HDL Counter : hdlsllib/Sources/HDL Counter  CountType=Count limited  CountInit=0  CountStep=1  CountMax=1  CountFromType=Initial value  CountFrom=0  CountResetPort=off  CountLoadPort=off  CountEnbPort=on  CountDirPort=off  CountHitOutputPort=off  CountDataType=Unsigned  CountWordLen=1  CountFracLen=0  CountSampTime=1
  Logical Operator : Logic  IconShape=distinctive  AllPortsSameDT=off  OutDataTypeStr=boolean
  Logical Operator1 : Logic  IconShape=distinctive  AllPortsSameDT=off  OutDataTypeStr=boolean
  Mux : Mux  Inputs=2
  Null : Constant  Value=complex(0,0)  OutDataTypeStr=fixdt(1,16,15)  SampleTime=1/(Rsym*SamplesPerSymbol)
  QPSK Modulator Baseband : commdigbbndpm3/QPSK Modulator Baseband  InType=Bit  Enc=Gray  Ph=pi/4  outDtype=Fixed-point  outWordLen=16  outUDDataType=sfix(16)  outFracLenMode=User-defined  outFracLen=15  outDataTypeStr=fixdt(1,16,15)  outLastDataTypeStr=fixdt(1,16,15)
  Switch3 : Switch  Threshold=1  SaturateOnIntegerOverflow=off  InputSameDT=off
  Unit Delay Enabled Synchronous : hdlsllib/Discrete/Unit Delay Enabled Synchronous  InitialCondition=0.0  SampleTime=-1
  dataOut : Outport
  validOut : Outport  Port=2
  wires:
  Delay5/1 -> Delay12/1
  Delay4/1 -> QPSK Modulator Baseband/1
  Mux/1 -> Delay4/1
  Unit Delay Enabled Synchronous/1 -> Mux/1
  Logical Operator/1 -> Unit Delay Enabled Synchronous/2
  Delay12/1 -> Delay3/1, Switch3/2
  Delay11/1 -> Switch3/1
  Compare To Constant1/1 -> Logical Operator1/1
  Compare To Constant/1 -> Logical Operator/2
  Delay1/1 -> HDL Counter/1, Logical Operator/1, Logical Operator1/2
  Delay3/1 -> validOut/1
  Delay2/1 -> dataOut/1
  Delay/1 -> Unit Delay Enabled Synchronous/1, Mux/2
  Null/1 -> Switch3/3
  Switch3/1 -> Delay2/1
  Logical Operator1/1 -> Delay5/1
  QPSK Modulator Baseband/1 -> Delay11/1
  HDL Counter/1 -> Compare To Constant1/1, Compare To Constant/1
  validIn/1 -> Delay1/1
  dataIn/1 -> Delay/1

== system commhdlQPSKTxRxLoopback/TxRxComposite/Transmitter/QPSK Tx/RRC Transmit Filter ==
  dataIn : Inport
  validIn : Inport  Port=2
  Data Type Conversion : DataTypeConversion  OutDataTypeStr=fixdt(1,17,16)  SaturateOnIntegerOverflow=off  RndMeth=Floor
  Data Type Conversion1 : DataTypeConversion  OutDataTypeStr=fixdt(1,16,14)  SaturateOnIntegerOverflow=off  RndMeth=Floor
  Delay1 : Delay  DelayLength=1
  Delay2 : Delay  DelayLength=1
  Delay3 : Delay  DelayLength=1
  RRC Filter : dsphdlfiltering2/Discrete FIR Filter  NumeratorSource=Property  Numerator=RRCCoef  NumeratorPrototype=[]  FilterStructure=Direct form systolic  SerializationOption=Minimum number of cycles between valid input samples  NumCycles=2  NumberOfMultipliers=2  SimulateUsing=Code generation  roundingMode=Floor  overflowMode=off  CoefficientsDataTypeStr=Inherit: Same word length as input  OutputDataTypeStr=Inherit: Same word length as input  ResetInputPort=off  HDLGlobalReset=off  CoeffMultiplier=Multiplier  UseMultForPow2Coeff=on  FrameInputSymmOptim=off
  Unit Delay Enabled Synchronous1 : hdlsllib/Discrete/Unit Delay Enabled Synchronous  InitialCondition=0  SampleTime=-1
  dataOut : Outport
  validOut : Outport  Port=2
  wires:
  Delay3/1 -> RRC Filter/1
  validIn/1 -> Unit Delay Enabled Synchronous1/1, Unit Delay Enabled Synchronous1/2
  Data Type Conversion1/1 -> Delay1/1
  Unit Delay Enabled Synchronous1/1 -> RRC Filter/2
  Data Type Conversion/1 -> Delay3/1
  Delay2/1 -> validOut/1
  Delay1/1 -> dataOut/1
  RRC Filter/2 -> Delay2/1
  RRC Filter/1 -> Data Type Conversion1/1
  dataIn/1 -> Data Type Conversion/1

== system commhdlQPSKTxRxLoopback/Receiver/QPSK Rx/Frequency and Time Synchronizer/Carrier Synchronizer/Direct Digital Synthesis ==
  rst : Inport
  validIn : Inport  Port=2
  phaseInc : Inport  Port=3
  Data Type Conversion : DataTypeConversion  OutDataTypeStr=fixdt(1,21,21)  SaturateOnIntegerOverflow=off  RndMeth=Floor
  Data Type Conversion1 : DataTypeConversion  OutDataTypeStr=fixdt(1,21,0)  ConvertRealWorld=Stored Integer (SI)  SaturateOnIntegerOverflow=off  RndMeth=Floor
  Delay : Delay  DelayLength=1
  NCO : dsphdlsigops2/NCO  PhaseIncrementSource=Input port  PhaseIncrement=0  PhaseOffsetSource=Property  PhaseOffset=0  DitherSource=Property  NumDitherBits=11  SamplesPerFrame=1  LUTCompress=off  ResetAction=on  Waveform=Complex exponential  PhasePort=off  SimulateUsing=Code generation  AccumulatorWL=21  PhaseQuantization=on  NumQuantizerAccumulatorBits=14  OutputDataType=Binary point scaling  OutputWL=16  OutputFL=14
  Terminator : Terminator
  expOut : Outport
  wires:
  Data Type Conversion/1 -> Data Type Conversion1/1
  NCO/1 -> expOut/1
  validIn/1 -> NCO/3
  Data Type Conversion1/1 -> NCO/1
  NCO/2 -> Terminator/1
  Delay/1 -> Data Type Conversion/1
  phaseInc/1 -> Delay/1
  rst/1 -> NCO/2

== system commhdlQPSKTxRxLoopback/Receiver/QPSK Rx/Frequency and Time Synchronizer/Carrier Synchronizer/Loop Filter ==
  e : Inport
  validIn : Inport  Port=2
  internalRst : Inport  Port=3
  externalRst : Inport  Port=4
  Add : Sum  Inputs=+|+
  Add1 : Sum  Inputs=|++  OutDataTypeStr=Inherit: Same as first input
  Data Type Conversion1 : DataTypeConversion  OutDataTypeStr=fixdt(1,29,29)  SaturateOnIntegerOverflow=off  RndMeth=Floor
  Data Type Conversion2 : DataTypeConversion  OutDataTypeStr=fixdt(1,39,39)  SaturateOnIntegerOverflow=off  RndMeth=Floor
  Delay : Delay  DelayLength=1
  Delay{1..11,13} (12 alike) : Delay
  Delay12 : Delay  DelayLength=1
  Gain : Gain  Gain=fi(CSLoopFilterIntegGain/(2*pi),0,16,16)  ParamDataTypeStr=Inherit: Inherit from 'Gain'
  Gain1 : Gain  Gain=fi(CSLoopFilterPropGain/(2*pi),0,16,16)  ParamDataTypeStr=Inherit: Inherit from 'Gain'
  Logical Operator : Logic  Operator=OR  AllPortsSameDT=off  OutDataTypeStr=boolean
  Unit Delay Enabled Resettable Synchronous : hdlsllib/Discrete/Unit Delay Enabled Resettable Synchronous  InitialCondition=0.0  SampleTime=-1
  Unit Delay Enabled Resettable Synchronous1 : hdlsllib/Discrete/Unit Delay Enabled Resettable Synchronous  InitialCondition=0.0  SampleTime=-1
  v : Outport
  valid : Outport  Port=2
  rst : Outport  Port=3
  wires:
  Delay6/1 -> Data Type Conversion1/1
  Delay5/1 -> Gain/1
  Delay7/1 -> Gain1/1
  Gain/1 -> Delay1/1
  Data Type Conversion2/1 -> Add1/1
  Delay3/1 -> Add/2
  Delay1/1 -> Data Type Conversion2/1
  Gain1/1 -> Delay6/1
  Delay2/1 -> Add/1
  Add/1 -> v/1
  e/1 -> Delay7/1, Delay5/1
  Data Type Conversion1/1 -> Unit Delay Enabled Resettable Synchronous/1
  Add1/1 -> Unit Delay Enabled Resettable Synchronous1/1
  Unit Delay Enabled Resettable Synchronous1/1 -> Delay3/1, Add1/2
  Unit Delay Enabled Resettable Synchronous/1 -> Delay2/1
  Logical Operator/1 -> Unit Delay Enabled Resettable Synchronous/3, Unit Delay Enabled Resettable Synchronous1/3
  validIn/1 -> Delay8/1
  Delay8/1 -> Delay4/1
  externalRst/1 -> Logical Operator/1
  internalRst/1 -> Delay9/1
  Delay9/1 -> Delay10/1
  Delay10/1 -> Delay12/1, Logical Operator/2
  Delay4/1 -> Unit Delay Enabled Resettable Synchronous/2, Unit Delay Enabled Resettable Synchronous1/2, Delay/1
  Delay11/1 -> valid/1
  Delay/1 -> Delay11/1
  Delay12/1 -> Delay13/1
  Delay13/1 -> rst/1

== system commhdlQPSKTxRxLoopback/Receiver/QPSK Rx/Frequency and Time Synchronizer/Carrier Synchronizer/Phase Error Detector ==
  dataIn : Inport
  Add : Sum  Inputs=+|-
  Compare To Constant : simulink/Logic and Bit Operations/Compare To Constant  relop=>=  const=0  OutDataTypeStr=boolean
  Compare To Constant1 : simulink/Logic and Bit Operations/Compare To Constant  relop=>=  const=0  OutDataTypeStr=boolean
  Complex to Real-Imag : ComplexToRealImag
  Constant : Constant  OutDataTypeStr=fixdt(1,2,0)  SampleTime=1/(Rsym*SamplesPerSymbol)
  Constant1 : Constant  Value=-1  OutDataTypeStr=fixdt(1,2,0)  SampleTime=1/(Rsym*SamplesPerSymbol)
  Constant2 : Constant  OutDataTypeStr=fixdt(1,2,0)  SampleTime=1/(Rsym*SamplesPerSymbol)
  Constant3 : Constant  Value=-1  OutDataTypeStr=fixdt(1,2,0)  SampleTime=1/(Rsym*SamplesPerSymbol)
  Data Type Conversion3 : DataTypeConversion  OutDataTypeStr=fixdt(1,10+3,10)  SaturateOnIntegerOverflow=off  RndMeth=Floor
  Delay{,1..6} (7 alike) : Delay
  Product : Product
  Product1 : Product
  Switch : Switch  Threshold=1  SaturateOnIntegerOverflow=off  InputSameDT=off
  Switch1 : Switch  Threshold=1  SaturateOnIntegerOverflow=off  InputSameDT=off
  PhaseError : Outport
  wires:
  Complex to Real-Imag/1 -> Delay2/1, Compare To Constant/1
  Compare To Constant1/1 -> Switch1/2
  Constant/1 -> Switch/1
  Constant3/1 -> Switch1/3
  Constant2/1 -> Switch1/1
  Constant1/1 -> Switch/3
  Compare To Constant/1 -> Switch/2
  Add/1 -> Delay6/1
  Switch/1 -> Delay/1
  Product1/1 -> Delay5/1
  Product/1 -> Delay4/1
  Switch1/1 -> Delay3/1
  Complex to Real-Imag/2 -> Delay1/1, Compare To Constant1/1
  dataIn/1 -> Complex to Real-Imag/1
  Delay/1 -> Product/1
  Delay1/1 -> Product/2
  Delay2/1 -> Product1/1
  Delay3/1 -> Product1/2
  Delay4/1 -> Add/1
  Delay5/1 -> Add/2
  Delay6/1 -> Data Type Conversion3/1
  Data Type Conversion3/1 -> PhaseError/1

== system commhdlQPSKTxRxLoopback/Receiver/QPSK Rx/Frequency and Time Synchronizer/Coarse Frequency Compensator/CFO step change detector ==
  note: fixed point precision loss warning supressed for this subsystem
  In1 : Inport
  Add : Sum  Inputs=+-
  Compare To Constant : simulink/Logic and Bit Operations/Compare To Constant  relop=>  const=fi(CFOChangeDetectThreshold,1,22,21)  OutDataTypeStr=boolean
  Compare To Constant1 : simulink/Logic and Bit Operations/Compare To Constant  relop=<  const=fi(-CFOChangeDetectThreshold,1,22,21)  OutDataTypeStr=boolean
  Delay : Delay  DelayLength=6
  Delay1 : Delay  DelayLength=1
  Logical Operator : Logic  Operator=OR  AllPortsSameDT=off  OutDataTypeStr=boolean
  Out1 : Outport
  wires:
  In1/1 -> Add/1, Delay1/1
  Delay/1 -> Out1/1
  Delay1/1 -> Add/2
  Add/1 -> Compare To Constant/1, Compare To Constant1/1
  Compare To Constant/1 -> Logical Operator/1
  Logical Operator/1 -> Delay/1
  Compare To Constant1/1 -> Logical Operator/2
